simulink model "unipolar_sim_PIL"  (R2026b)
settings: Solver=VariableStepAuto  StopTime=2
undefined symbols (not defined in the file): L, PWM_mode, T_threshold, Tpwm, Vmax
libraries: fl_lib x11, nesl_utility x8, ee_lib x4, eeGeneralControl x4, sl_discontinuities x2, simulink x1
settings Model: Creator=Samuel  LastModifiedBy=Samuel
settings SimscapeCC: SimscapeUseEnergyAccounting=off

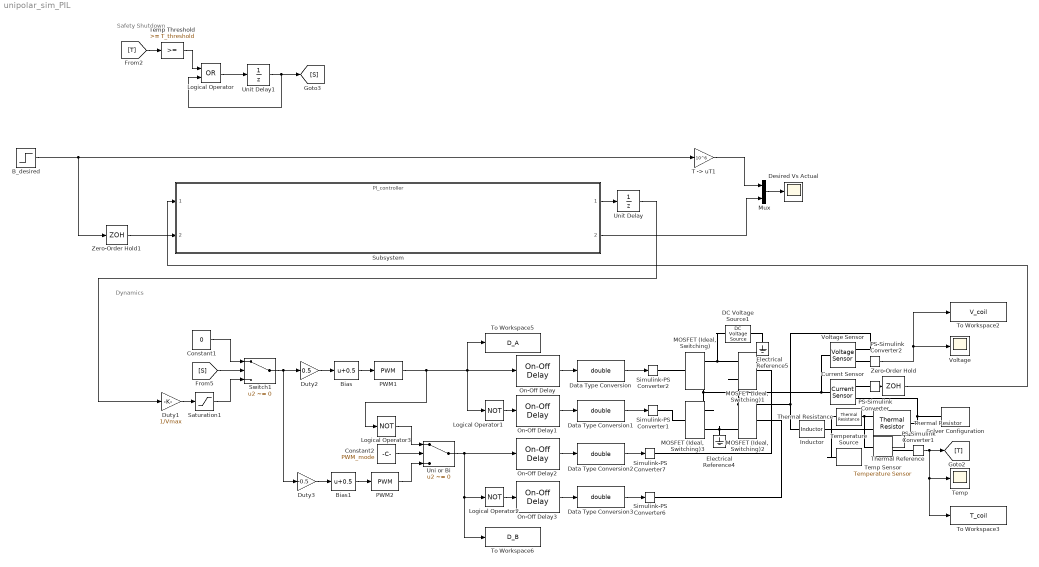
== system unipolar_sim_PIL ==
  note: Dynamics
  note: Safety Shutdown
  B_desired : Step  Time=0.3  InitialValue=100e-6  FinalValue=-100e-6  SampleTime=0
  Bias : Bias  Bias=0.5  SaturateOnIntegerOverflow=off
  Bias1 : Bias  Bias=0.5  SaturateOnIntegerOverflow=off
  Constant1 : Constant  Value=0
  Constant2 : Constant  Value=PWM_mode
  Current Sensor : fl_lib/Electrical/Electrical Sensors/Current Sensor
  DC Voltage Source1 : fl_lib/Electrical/Electrical Sources/DC Voltage Source  v0=[Vmax] V
  Data Type Conversion{,1..3} (4 alike) : DataTypeConversion  OutDataTypeStr=double  SaturateOnIntegerOverflow=off  RndMeth=Floor
  Desired Vs Actual : Scope
      settings: ActiveDisplayYMinimum=-149.18256789839177  ActiveDisplayYMaximum=155.95150192959457  DataLoggingMaxPoints=1000000000
  Duty1 : Gain  Gain=1/Vmax
  Duty2 : Gain  Gain=0.5
  Duty3 : Gain  Gain=-0.5
  Electrical Reference4 : fl_lib/Electrical/Electrical Elements/Electrical Reference
  Electrical Reference5 : fl_lib/Electrical/Electrical Elements/Electrical Reference
  Inductor : fl_lib/Electrical/Electrical Elements/Inductor  l=[L] H  r=0 Ohm  g=1e-9 1/Ohm  i_specify=off  i_priority=None  i=0 A  i_nominal_specify=off  i_nominal_value=1  i_nominal_unit=A  v_specify=off  v_priority=None  v=0 V  v_nominal_specify=off  v_nominal_value=1  v_nominal_unit=V  i_L_specify=off  i_L_priority=High  i_L=0 A  i_L_nominal_specify=off  i_L_nominal_value=1  i_L_nominal_unit=A
  Logical Operator : Logic  Operator=OR  AllPortsSameDT=off  OutDataTypeStr=boolean
  Logical Operator1 : Logic  Operator=NOT  AllPortsSameDT=off  OutDataTypeStr=boolean
  Logical Operator2 : Logic  Operator=NOT  AllPortsSameDT=off  OutDataTypeStr=boolean
  Logical Operator3 : Logic  Operator=NOT  AllPortsSameDT=off  OutDataTypeStr=boolean
  MOSFET (Ideal, Switching){,1..3} (4 alike) : ee_lib/Semiconductors & Converters/MOSFET (Ideal, Switching)  port_option=ee.enum.controlport.ps  Rds=0.01 Ohm  Goff=1e-6 1/Ohm  Vth=0.5 V  diode_param=ee.enum.converters.protectiondiode.nodynamics  diode_Vf=0.8 V  diode_Ron=0.001 Ohm  diode_Goff=1e-5 1/Ohm  diode_C=50e-9 F  diode_iRM=-235 A  diode_iF=300 A  diode_idot=-50 A/us  diode_trr_param=ee.enum.converters.diodeReverseParam.trr_factor  diode_trr_factor=3  diode_trr=15 us  diode_Qrr=1500 s*uA  ids_specify=off  ids_priority=None  ids=0 A  ids_nominal_specify=off  ids_nominal_value=1  ids_nominal_unit=A  vds_specify=off  vds_priority=None  vds=0 V  vds_nominal_specify=off  vds_nominal_value=1  vds_nominal_unit=V  vgs_specify=off  vgs_priority=None  vgs=0 V  vgs_nominal_specify=off  vgs_nominal_value=1  vgs_nominal_unit=V  thermal_loss_option=ee.enum.converters.thermalLossOption.constantvalues  Von_data=[0, 1.8, 3.2, 6, 10, 16; 0, 2, 5.5, 9.5, 15, 25] V  Tj=[298.15, 448.15] K  Iout_data=[0, 20, 40, 60, 80, 100] A  tabulateWithVds=false  Eon_data=[0, 55.04, 124.57, 235.53, 362.12; 0, 71.25, 161.25, 304.88, 468.75] * 1e-6 J  Eoff_data=[0, 18, 30, 56.1, 76.5; 0, 22.5, 37.5, 70.13, 95.63] * 1e-6 J  Eon_data_3D=[zeros(2, 5, 3)] J  Eoff_data_3D=[zeros(2, 5, 3)] J  Tj_loss=[298.15, 448.15] K  Iout_data_loss=[0, 10, 20, 30, 40] A  Vds_loss=[0, 150, 300] V  Eon_scalar=22.86e-3 J  Eoff_scalar=17.14e-3 J  Voff=300 V  Iout_scalar=600 A  useCurrentFromPreviousCycle=false  currentMeasDelay=0 s  useVoltageFromPreviousCycle=false  voltageMeasDelay=0 s  diodeModelType=ee.enum.converters.diodeModelType.pwl  diodeTableType=ee.enum.diode.tableType.IfMat  diode_ReverseIVType=ee.enum.diode.diodeReverseIV.constant  diode_IfMat=[.07, .12, .19, 1.75, 4.24, 7.32, 11.2; .16, .3, .72, 2.14, 4.02, 6.35, 9.12] A  diode_VfMat=[.9, 1.15, 1.25, 1.5, 1.75, 2.17, 2.6, 2.85; .58, .68, .75, 1.1, 1.38, 1.77, 2.27, 2.7] V  diode_TjVec=[25, 125] degC  diode_VfVec=[.5, .7, .9, 1.3, 1.7, 2.1, 2.5] V  diode_IfVec=[.1, .2, .5, 1, 2, 4, 7, 10] A  diode_IrMat=[1e-06, 2e-06, 5e-06, 1e-05, 2.5e-05, 5e-05, .0001; 2e-06, 5e-06, 1e-05, 4e-05, 8e-05, .0002, .0005] A  diode_VrMat=[10, 100, 200, 250, 300, 325, 350; 10, 70, 160, 220, 270, 300, 320] V  diode_VrVec=[10, 20, 40, 50, 70, 80, 100] V  diode_IrVec=[1e-06, 2e-06, 5e-06, 1e-05, 2e-05, 5e-05, .0001] A  diode_Vr=-600 V  diode_Ls=150 nH  diode_Erec=0.03 J  diode_rec_loss_model=ee.enum.diode.reverseRecoveryModel.fixed  diode_ErecVal=0 J  diode_scaleWithIandV=true  diode_ErecMat=zeros(2, 3) J  diodeErecMat3D=zeros(2, 3, 2) J  diode_TjrecVec=[298.15, 398.15] K  diode_IfrecVec=[.1, 1, 10] A  diodeVrecVec=[0, 100] V  diode_IrecVal=10 A  diode_VrecVal=10 V  diode_tFilter=1 / 1000 / 100 s  separateThermalPortForDiode=false  thermal_network_parameterization=ee.enum.thermalNetworkTopology.external  Rth=[.03, .2] K/W  Rth_Cauer=[.03, .1, .2] K/W  Rth_Foster=[.03, .2] K/W  thermal_mass_parameterization=ee.enum.thermalNetwork.timeconstant  thermal_mass=[3, 25] J/K  thermal_mass_Cauer=[3, 10, 25] J/K  thermal_mass_Foster=[33, 50] J/K  thermal_time_constant=[.1, 5] s  thermal_time_constant_Cauer=[.1, 1, 5] s  thermal_time_constant_Foster=[1, 10] s  thermal_mass_initial_temperatures=[25, 25] degC  thermal_mass_initial_temperatures_Cauer=[25, 25, 25] degC  junction_thermal_mass=0.1 J/K  Tvec_initial_Foster=[25, 25, 25, 25] degC  RthDiode=[.03, .2] K/W  RthCauerDiode=[.03, .1, .2] K/W  RthFosterDiode=[.03, .2] K/W  thermalMassDiode=[3, 25] J/K  thermalMassCauerDiode=[3, 10, 25] J/K  thermalMassFosterDiode=[33, 50] J/K  thermalTauDiode=[.1, 5] s  thermalTauCauerDiode=[.1, 1, 5] s  thermalTauFosterDiode=[1, 10] s  thermalMassInitTempDiode=[25, 25] degC  thermalMassInitTempCauerDiode=[25, 25, 25] degC  junctionthermalMassDiode=0.1 J/K  TVecInitialFosterDiode=[25, 25] degC  no_thermal_network=0  mosfet_junction_temperature_specify=off  mosfet_junction_temperature_priority=None  mosfet_junction_temperature=25 degC  mosfet_junction_temperature_nominal_specify=off  mosfet_junction_temperature_nominal_value=1  mosfet_junction_temperature_nominal_unit=degC  diode_junction_temperature_specify=off  diode_junction_temperature_priority=None  diode_junction_temperature=25 degC  diode_junction_temperature_nominal_specify=off  diode_junction_temperature_nominal_value=1  diode_junction_temperature_nominal_unit=degC  Qj_specify=off  Qj_priority=None  Qj=0 W  Qj_nominal_specify=off  Qj_nominal_value=1  Qj_nominal_unit=W  accumulatedSwitchingLosses_specify=off  accumulatedSwitchingLosses_priority=None  accumulatedSwitchingLosses=0 J
  Mux : Mux  Inputs=2
  On-Off Delay{,1..3} (4 alike) : eeGeneralControl/On-Off Delay  LabelModeActiveChoice=Continuous  Td_on=t_dead  Td_off=0  IC=0  Ts=0
      settings: LibrarySourceBlock=ee_sl_lib/General Control/On-Off Delay
  PS-Simulink Converter : nesl_utility/PS-Simulink Converter  PhysicalDomain=network_engine_domain  SubClassName=ps_output  LeftPortType=input  RightPortType=output  PseudoPeriodic=off  Frequencies=[]  VectorFormat=inherit  Unit=inherit  AffineConversion=off
  PS-Simulink Converter1 : nesl_utility/PS-Simulink Converter  PhysicalDomain=network_engine_domain  SubClassName=ps_output  LeftPortType=input  RightPortType=output  PseudoPeriodic=off  Frequencies=[]  VectorFormat=inherit  Unit=inherit  AffineConversion=off
  PS-Simulink Converter2 : nesl_utility/PS-Simulink Converter  PhysicalDomain=network_engine_domain  SubClassName=ps_output  LeftPortType=input  RightPortType=output  PseudoPeriodic=off  Frequencies=[]  VectorFormat=inherit  Unit=inherit  AffineConversion=off
  PWM1 : sl_discontinuities/PWM  DisableCoverage=on  Period=[Tpwm]  InitialDelay=0  DisallowZeroDutyCycle=off  RunAtFixedTimeIntervals=off  SampleTime=0.1
  PWM2 : sl_discontinuities/PWM  DisableCoverage=on  Period=[Tpwm]  InitialDelay=0  DisallowZeroDutyCycle=off  RunAtFixedTimeIntervals=off  SampleTime=0.1
  Saturation1 : Saturate  UpperLimit=1  LowerLimit=-1
  Simulink-PS Converter{1..2,6..7} (4 alike) : nesl_utility/Simulink-PS Converter  PhysicalDomain=network_engine_domain  SubClassName=ps_input  LeftPortType=input  RightPortType=output  PseudoPeriodic=off  Frequencies=[]  NoiseDistribution=none  NoiseParameters=[]  Unit=1  AffineConversion=off  FilteringAndDerivatives=provide  SimscapeFilterOrder=1  InputFilterTimeConstant=0.001  UdotUserProvided=0
  Solver Configuration : nesl_utility/Solver Configuration  PhysicalDomain=network_engine_domain  SubClassName=solver  LeftPortType=input  RightPortType=generic  Tones=[]  Harmonics=[]  SimulateNoise=off  Profile=off  UseLocalSampling=off  EnableSwitchedLinearOptims=on  FrequencyDomain=off  UseCCode=off  RelTol=0.001  AbsTol=0.001  MinStep=1e-09  ToWorkspace=off  RevertToSquareIcSolve=off  NumHomotopyIterations=100  PhasorMode=off  PhasorModeNumHarmonics=1  ConsistencySolver=NEWTON_XTOL_AFTER_FTOL  CanonicalOrdering=UNORDERED  OptimizeIntermediates=UNOPTIMIZED  MulticoreSolverChoice=BACKWARD_EULER  IndexReductionMethod=DerivativeReplacement  DoDC=off  ResidualTolerance=1e-09  ConsistencyTolSource=GLOBAL  ConsistencyAbsTol=0.001  ConsistencyRelTol=0.001  ConsistencyTolFactor=0.001  UseLocalSolver=off  LocalSolverChoice=NE_BACKWARD_EULER_ADVANCER  ResolveIndetEquations=on  FunctionEvalNumThread=1  LocalSolverSampleTime=0.001  DoFixedCost=off  MaxNonlinIter=3  MaxModeIter=2  ComputeImpulses=off  ImpulseIterations=2  LinearAlgebra=auto  LinearAlgebraNumThread=0  EquationFormulation=NE_TIME_EF  DelaysMemoryBudget=1024  AutomaticFiltering=on  FilteringTimeConstant=0.001  PartitionStorageMethod=AS_NEEDED  PartitionMemoryBudget=1024  PartitionMethod=BALANCED  MultibodyUseLocalSolver=off  MultibodyLocalSolverChoice=ODE1  MultibodyLocalSolverSampleTime=0.001
  Subsystem : ModelReference  ModelNameDialog=PI_controller  SimulationMode=Processor-in-the-loop (PIL)  ModelReferenceVersion=7.10
  Switch1 : Switch  Criteria=u2 ~= 0  SaturateOnIntegerOverflow=off  InputSameDT=off
  "T -> uT1" : Gain  Gain=10^6
  Temp : Scope
      settings: ActiveDisplayYMinimum=293.07345  ActiveDisplayYMaximum=293.83895  DataLoggingVariableName=ScopeData2
  Temp Threshold : simulink/Logic and Bit Operations/Compare To Constant  relop=>=  const=T_threshold  OutDataTypeStr=boolean
  Temp Sensor : fl_lib/Thermal/Thermal Sensors/Temperature Sensor  temperature_measure=foundation.enum.MeasurementReference.difference
  Temperature Source : fl_lib/Thermal/Thermal Sources/Temperature Source  temperature=293.15 K
  Thermal Reference : fl_lib/Thermal/Thermal Elements/Thermal Reference
  Thermal Resistance : fl_lib/Thermal/Thermal Elements/Thermal Resistance  resistance=R_th K/W  T_specify=off  T_priority=None  T=0 K  T_nominal_specify=off  T_nominal_value=1  T_nominal_unit=K  Q_specify=off  Q_priority=None  Q=0 W  Q_nominal_specify=off  Q_nominal_value=1  Q_nominal_unit=W
  Thermal Resistor : fl_lib/Electrical/Electrical Elements/Thermal Resistor  R0=R_coil_ref Ohm  T0=T_coil_ref K  alpha=alpha_coil 1/K  thermalMassParameterization=foundation.enum.ThermalMassParameterization.TimeConstantAndDissipationFactor  mass=2.6316e-5 kg  cp=380 J/(K*kg)  tc=tau_coil_th s  K_d=G_coil_loss W/K  T_specify=on  T_priority=High  T=293.15 K  T_nominal_specify=off  T_nominal_value=1  T_nominal_unit=K
  To Workspace2 : ToWorkspace  VariableName=V_coil  SaveFormat=Timeseries  SampleTime=-1
  To Workspace3 : ToWorkspace  VariableName=T_coil  SaveFormat=Timeseries  SampleTime=-1
  To Workspace5 : ToWorkspace  VariableName=D_A  SaveFormat=Timeseries  SampleTime=-1
  To Workspace6 : ToWorkspace  VariableName=D_B  SaveFormat=Timeseries  SampleTime=-1
  Uni or Bi : Switch  Criteria=u2 ~= 0  SaturateOnIntegerOverflow=off  InputSameDT=off
  Unit Delay : UnitDelay  SampleTime=1e-4
  Unit Delay1 : UnitDelay  SampleTime=1e-4
  Voltage : Scope
      settings: ActiveDisplayYMinimum=-32.004329008257642  ActiveDisplayYMaximum=32.005813602780151
  Voltage Sensor : fl_lib/Electrical/Electrical Sensors/Voltage Sensor
  Zero-Order Hold : ZeroOrderHold  SampleTime=1e-4
  Zero-Order Hold1 : ZeroOrderHold  SampleTime=1e-4
  wires:
  Mux/1 -> Desired Vs Actual/1
  Temp Threshold/1 -> Logical Operator/1
  PS-Simulink Converter1/1 -> [T], To Workspace3/1, Temp/1
  [T] -> Temp Threshold/1
  Unit Delay1/1 -> Logical Operator/2, [S]
  Logical Operator/1 -> Unit Delay1/1
  Duty2/1 -> Bias/1
  Bias/1 -> PWM1/1
  PWM1/1 -> Logical Operator3/1, On-Off Delay/1, To Workspace5/1, Logical Operator1/1
  Uni or Bi/1 -> On-Off Delay2/1, To Workspace6/1, Logical Operator2/1
  Switch1/1 -> Duty2/1, Duty3/1
  [S] -> Switch1/2
  Constant1/1 -> Switch1/1
  Saturation1/1 -> Switch1/3
  Duty1/1 -> Saturation1/1
  PS-Simulink Converter2/1 -> Voltage/1, To Workspace2/1
  On-Off Delay2/1 -> Data Type Conversion2/1
  On-Off Delay/1 -> Data Type Conversion/1
  Data Type Conversion2/1 -> Simulink-PS Converter7/1
  Data Type Conversion3/1 -> Simulink-PS Converter6/1
  Data Type Conversion1/1 -> Simulink-PS Converter1/1
  Data Type Conversion/1 -> Simulink-PS Converter2/1
  Duty3/1 -> Bias1/1
  Bias1/1 -> PWM2/1
  Logical Operator3/1 -> Uni or Bi/1
  PWM2/1 -> Uni or Bi/3
  Constant2/1 -> Uni or Bi/2
  On-Off Delay1/1 -> Data Type Conversion1/1
  Logical Operator1/1 -> On-Off Delay1/1
  On-Off Delay3/1 -> Data Type Conversion3/1
  Logical Operator2/1 -> On-Off Delay3/1
  "T -> uT1"/1 -> Mux/1
  B_desired/1 -> "T -> uT1"/1, Zero-Order Hold1/1
  Subsystem/2 -> Mux/2
  PS-Simulink Converter/1 -> Zero-Order Hold/1
  Zero-Order Hold/1 -> Subsystem/1
  Zero-Order Hold1/1 -> Subsystem/2
  Subsystem/1 -> Unit Delay/1
  Unit Delay/1 -> Duty1/1
  connections:
  PS-Simulink Converter/LConn1 -- Current Sensor/RConn1
  Thermal Resistor/LConn2 -- Inductor/LConn1
  Thermal Resistor/LConn1 -- Thermal Resistance/LConn1 -- Temp Sensor/LConn1
  Temperature Source/LConn1 -- Thermal Resistance/RConn1
  Temp Sensor/RConn1 -- Thermal Reference/LConn1
  Thermal Resistor/RConn1 -- Solver Configuration/RConn1 -- Current Sensor/RConn2
  PS-Simulink Converter1/LConn1 -- Temp Sensor/RConn2
  "MOSFET (Ideal, Switching)3"/RConn2 -- Electrical Reference4/LConn1 -- "MOSFET (Ideal, Switching)2"/RConn2
  "MOSFET (Ideal, Switching)"/RConn1 -- DC Voltage Source1/LConn1 -- "MOSFET (Ideal, Switching)1"/RConn1
  "MOSFET (Ideal, Switching)3"/RConn1 -- Current Sensor/LConn1 -- Voltage Sensor/LConn1 -- "MOSFET (Ideal, Switching)"/RConn2
  "MOSFET (Ideal, Switching)1"/RConn2 -- "MOSFET (Ideal, Switching)2"/RConn1 -- Voltage Sensor/RConn2 -- Inductor/RConn1
  Electrical Reference5/LConn1 -- DC Voltage Source1/RConn1
  Voltage Sensor/RConn1 -- PS-Simulink Converter2/LConn1
  Simulink-PS Converter2/RConn1 -- "MOSFET (Ideal, Switching)"/LConn1
  Simulink-PS Converter1/RConn1 -- "MOSFET (Ideal, Switching)3"/LConn1
  Simulink-PS Converter7/RConn1 -- "MOSFET (Ideal, Switching)1"/LConn1
  Simulink-PS Converter6/RConn1 -- "MOSFET (Ideal, Switching)2"/LConn1
